simulink model "stage5i_secondary_test_harness"  (R2018b)
settings: Solver=FixedStepDiscrete  StartTime=0.0  StopTime=0.6  FixedStep=0.0001  RelTol=1e-3
model workspace (MAT data in the model file):
  frequency_test_signal = [0  313.530946828; 0.6  313.530946828]
  secondary_Ki = 4
  secondary_Ts = 0.0001
  secondary_enable = 1
  secondary_enable_time = 0.5
  secondary_f_ref_Hz = 50
  secondary_max_pu = 0.8
  secondary_min_pu = -0.5
undefined symbols (not defined in the file): DiscIntNeverNeededParam
settings Model: Creator=User  LastModifiedBy=User
settings DataIOCC: ReturnWorkspaceOutputs=on

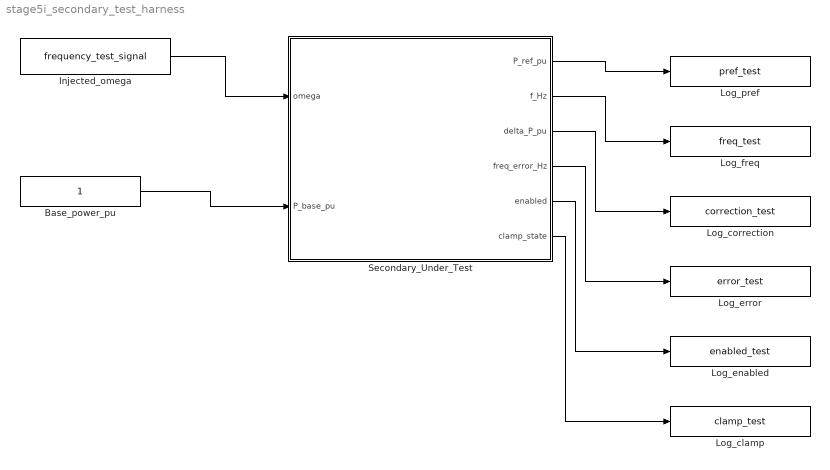
== system stage5i_secondary_test_harness ==
  Base_power_pu : Constant
  Injected_omega : FromWorkspace  VariableName=frequency_test_signal  Interpolate=off  OutputAfterFinalValue=Holding final value
  Log_clamp : ToWorkspace  VariableName=clamp_test  SaveFormat=Timeseries
  Log_correction : ToWorkspace  VariableName=correction_test  SaveFormat=Timeseries
  Log_enabled : ToWorkspace  VariableName=enabled_test  SaveFormat=Timeseries
  Log_error : ToWorkspace  VariableName=error_test  SaveFormat=Timeseries
  Log_freq : ToWorkspace  VariableName=freq_test  SaveFormat=Timeseries
  Log_pref : ToWorkspace  VariableName=pref_test  SaveFormat=Timeseries
  Secondary_Under_Test : Subsystem
  wires:
  Injected_omega/1 -> Secondary_Under_Test/1(omega)
  Base_power_pu/1 -> Secondary_Under_Test/2(P_base_pu)
  Secondary_Under_Test/1(P_ref_pu) -> Log_pref/1
  Secondary_Under_Test/2(f_Hz) -> Log_freq/1
  Secondary_Under_Test/3(delta_P_pu) -> Log_correction/1
  Secondary_Under_Test/4(freq_error_Hz) -> Log_error/1
  Secondary_Under_Test/5(enabled) -> Log_enabled/1
  Secondary_Under_Test/6(clamp_state) -> Log_clamp/1

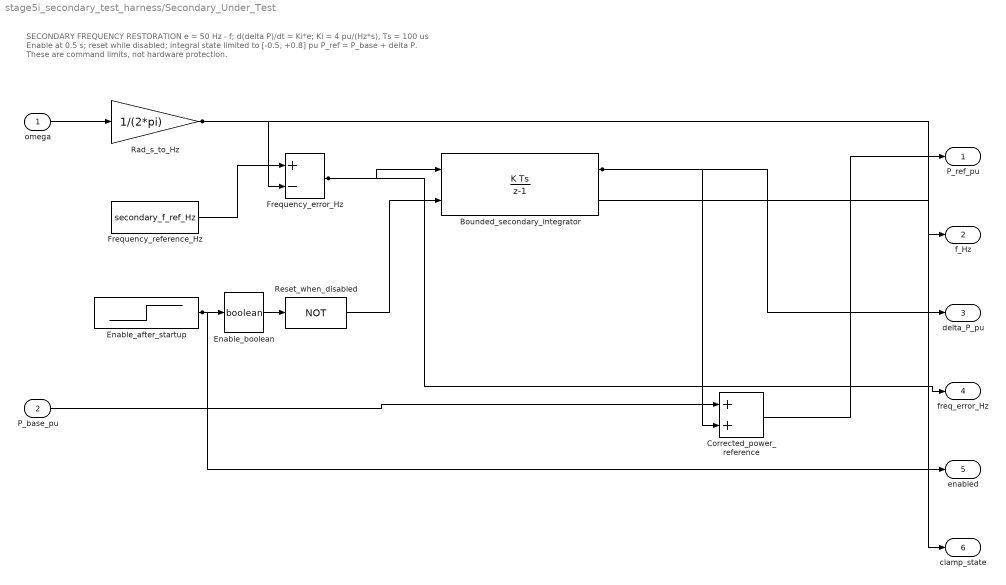
== system stage5i_secondary_test_harness/Secondary_Under_Test ==
  note: SECONDARY FREQUENCY RESTORATION
      | e = 50 Hz - f; d(delta P)/dt = Ki*e; Ki = 4 pu/(Hz*s), Ts = 100 us
      | Enable at 0.5 s; reset while disabled; integral state limited to [-0.5, +0.8] pu
      | P_ref = P_base + delta P. These are command limits, not hardware protection.
  omega : Inport
  P_base_pu : Inport  Port=2
  Bounded_secondary_integrator : DiscreteIntegrator  gainval=secondary_Ki  ExternalReset=level  SampleTime=secondary_Ts  LimitOutput=on  UpperSaturationLimit=secondary_max_pu  LowerSaturationLimit=secondary_min_pu  ShowSaturationPort=on  ICPrevOutput=DiscIntNeverNeededParam  ICPrevScaledInput=DiscIntNeverNeededParam
  Corrected_power_reference : Sum  SaturateOnIntegerOverflow=on  InputSameDT=on  OutDataTypeStr=Inherit: Same as first input
  Enable_after_startup : Step  Time=secondary_enable_time  After=secondary_enable  SampleTime=secondary_Ts
  Enable_boolean : DataTypeConversion  OutDataTypeStr=boolean  SaturateOnIntegerOverflow=on  RndMeth=Zero
  Frequency_error_Hz : Sum  Inputs=+-  SaturateOnIntegerOverflow=on  InputSameDT=on  OutDataTypeStr=Inherit: Same as first input
  Frequency_reference_Hz : Constant  Value=secondary_f_ref_Hz
  Rad_s_to_Hz : Gain  Gain=1/(2*pi)  SaturateOnIntegerOverflow=on  OutDataTypeStr=Inherit: Same as input  ParamDataTypeStr=Inherit: Same as input
  Reset_when_disabled : Logic  Operator=NOT
  P_ref_pu : Outport
  f_Hz : Outport  Port=2
  delta_P_pu : Outport  Port=3
  freq_error_Hz : Outport  Port=4
  enabled : Outport  Port=5
  clamp_state : Outport  Port=6
  wires:
  Bounded_secondary_integrator/2 -> clamp_state/1
  Corrected_power_reference/1 -> P_ref_pu/1
  Bounded_secondary_integrator/1 -> delta_P_pu/1, Corrected_power_reference/2
  P_base_pu/1 -> Corrected_power_reference/1
  Reset_when_disabled/1 -> Bounded_secondary_integrator/2
  Frequency_error_Hz/1 -> freq_error_Hz/1, Bounded_secondary_integrator/1
  Enable_boolean/1 -> Reset_when_disabled/1
  Enable_after_startup/1 -> enabled/1, Enable_boolean/1
  Rad_s_to_Hz/1 -> f_Hz/1, Frequency_error_Hz/2
  Frequency_reference_Hz/1 -> Frequency_error_Hz/1
  omega/1 -> Rad_s_to_Hz/1
